simulink library "Damper_Linear"  (R2025a)
settings: Solver=VariableStepAuto  StartTime=0.0  StopTime=10.0  RelTol=1e-3
undefined symbols (not defined in the file): Damper
libraries: fl_lib x5, nesl_utility x4
Description:
  | Component of Simscape Vehicle Templates Library
  | 
  | Copyright 2018-2026 The MathWorks, Inc.
settings Model: Creator=smiller  LastModifiedBy=smiller
settings SolverCC: AlgebraicLoopSolver=TrustRegion
settings DataIOCC: ReturnWorkspaceOutputs=off
settings OptimizationCC: ReuseModelBlockBuffer=off
settings DebuggingCC: UnconnectedInputMsg=warning  UnconnectedOutputMsg=warning  UnconnectedLineMsg=warning  ArithmeticOperatorsInVariantConditions=warning
settings ModelReferenceCC: EnableRefExpFcnMdlSchedulingChecks=on
settings SFSimCC: CustomCodeUndefinedFunction=UseInterfaceOnly
settings RTWCC: GPUComputeCapability=3.5  DLArmComputeVersion=19.05

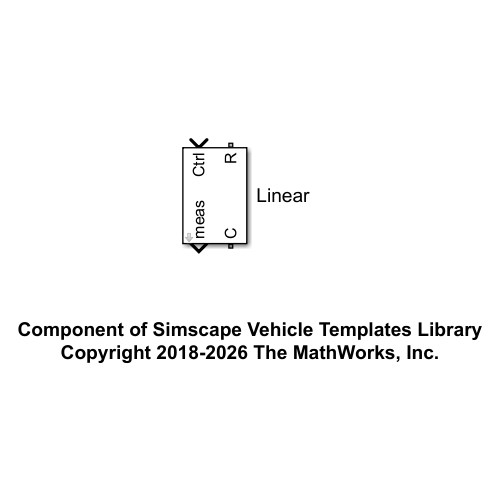
[thumbnail: Simulink's stored preview of the top-level diagram]
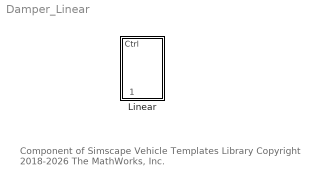
== system Damper_Linear ==
  note: Component of Simscape Vehicle Templates Library
      | Copyright 2018-2026 The MathWorks, Inc.
  Linear : Subsystem  VariantControl=Linear  mask(Linear Damper with Bumpstop){dam_b=Damper.Damping.d.Value, hp_dpr_top=Damper.Damping.sTop.Value, hp_dpr_bot=Damper.Damping.sBottom.Value, bs_lim_upper=Damper.Endstop.xMax.Value, bs_lim_lower=Damper.Endstop.xMin.Value, bs_k_upper=Damper.Endstop.KxMax.Value, bs_k_lower=Damper.Endstop.KxMin.Value, bs_b_upper=Damper.Endstop.dxMax.Value, bs_b_lower=Damper.Endstop.dxMin.Value, bs_region=Damper.Endstop.xTransition.Value}
      mask prompts: dam_b "Damper (N/(m/s))"; hp_dpr_top "HP Damper Top [xyz] (m)"; hp_dpr_bot "HP Damper Bottom [xyz] (m)"; bs_region "Transition Region (m)"
      mask help: Linear damper with bumpstop at top and bottom.
      mask init:
      | dam_x0 = norm(hp_dpr_top - hp_dpr_bot);
      mask TypeOptions dam_b: Damper/D
      mask DialogControl text_bumpstop_upper Prompt: Upper
      mask DialogControl text_bumpstop_lower Prompt: Lower
      mask DialogControl text_bumpstop_limit Prompt: Limit (m)
      mask DialogControl text_bumpstop_k Prompt: Stiffness (N/m)
      mask DialogControl text_bumpstop_b Prompt: Damping  (N/(m/s))

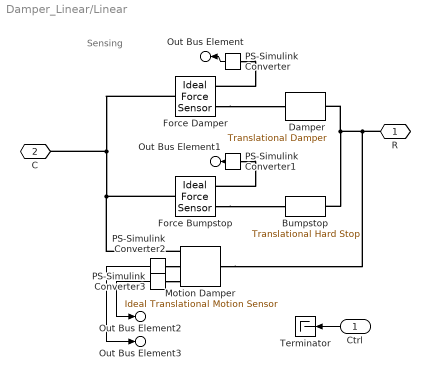
== system Damper_Linear/Linear ==
  note: Sensing
  Ctrl : Inport
  Bumpstop : fl_lib/Mechanical/Translational Elements/Translational Hard Stop  upper_bnd=bs_lim_upper m  lower_bnd=bs_lim_lower m  model=1  stiff_up=bs_k_upper N/m  stiff_low=bs_k_lower N/m  D_up=bs_b_upper N/(m/s)  D_low=bs_b_lower N/(m/s)  transition=bs_region m  coeff_rest=0.7  v_tol=0.001 m/s  f_tol=0.001 N  v_specify=off  v_priority=None  v=0 m/s  v_nominal_specify=off  v_nominal_value=1  v_nominal_unit=m/s  f_specify=off  f_priority=None  f=0 N  f_nominal_specify=off  f_nominal_value=1  f_nominal_unit=N  x_specify=off  x_priority=High  x=0 m  x_nominal_specify=off  x_nominal_value=1  x_nominal_unit=m  M_specify=off  M_priority=None  M=0
  Damper : fl_lib/Mechanical/Translational Elements/Translational Damper  D=dam_b N/(m/s)  v_specify=off  v_priority=None  v=0 m/s  v_nominal_specify=off  v_nominal_value=1  v_nominal_unit=m/s  f_specify=off  f_priority=None  f=0 N  f_nominal_specify=off  f_nominal_value=1  f_nominal_unit=N
  Force Bumpstop : fl_lib/Mechanical/Mechanical Sensors/Ideal Force Sensor
  Force Damper : fl_lib/Mechanical/Mechanical Sensors/Ideal Force Sensor
  Motion Damper : fl_lib/Mechanical/Mechanical Sensors/Ideal Translational Motion Sensor  reference=foundation.enum.MeasurementReference.difference  acceleration_port=false  velocity_port=true  position_port=true  offset=dam_x0 m
  PS-Simulink Converter : nesl_utility/PS-Simulink Converter  PhysicalDomain=network_engine_domain  SubClassName=ps_output  LeftPortType=input  RightPortType=output  PseudoPeriodic=off  Frequencies=[]  VectorFormat=1-D array  Unit=N  AffineConversion=off
  PS-Simulink Converter1 : nesl_utility/PS-Simulink Converter  PhysicalDomain=network_engine_domain  SubClassName=ps_output  LeftPortType=input  RightPortType=output  PseudoPeriodic=off  Frequencies=[]  VectorFormat=1-D array  Unit=N  AffineConversion=off
  PS-Simulink Converter2 : nesl_utility/PS-Simulink Converter  PhysicalDomain=network_engine_domain  SubClassName=ps_output  LeftPortType=input  RightPortType=output  PseudoPeriodic=off  Frequencies=[]  VectorFormat=1-D array  Unit=m/s  AffineConversion=off
  PS-Simulink Converter3 : nesl_utility/PS-Simulink Converter  PhysicalDomain=network_engine_domain  SubClassName=ps_output  LeftPortType=input  RightPortType=output  PseudoPeriodic=off  Frequencies=[]  VectorFormat=1-D array  Unit=m  AffineConversion=off
  Terminator : Terminator
  R : PMIOPort  Side=Left
  C : PMIOPort  Port=2  Side=Right
  Out Bus Element : Outport  VectorParamsAs1DForOutWhenUnconnected=off  PortName=meas  Element=FDamper
  Out Bus Element1 : Outport  VectorParamsAs1DForOutWhenUnconnected=off  PortName=meas  Element=FBumpstop
  Out Bus Element2 : Outport  VectorParamsAs1DForOutWhenUnconnected=off  PortName=meas  Element=xDamper
  Out Bus Element3 : Outport  VectorParamsAs1DForOutWhenUnconnected=off  PortName=meas  Element=vDamper
  wires:
  Ctrl/1 -> Terminator/1
  PS-Simulink Converter/1 -> Out Bus Element/1
  PS-Simulink Converter2/1 -> Out Bus Element3/1
  PS-Simulink Converter3/1 -> Out Bus Element2/1
  PS-Simulink Converter1/1 -> Out Bus Element1/1
  connections:
  Motion Damper/RConn1 -- Force Bumpstop/LConn1 -- C/RConn1 -- Force Damper/LConn1
  PS-Simulink Converter2/LConn1 -- Motion Damper/RConn2
  PS-Simulink Converter1/LConn1 -- Force Bumpstop/RConn2
  PS-Simulink Converter3/LConn1 -- Motion Damper/RConn3
  PS-Simulink Converter/LConn1 -- Force Damper/RConn2
  Force Bumpstop/RConn1 -- Bumpstop/RConn1
  Force Damper/RConn1 -- Damper/RConn1
  Damper/LConn1 -- Bumpstop/LConn1 -- Motion Damper/LConn1 -- R/RConn1
